simulink model "test_locked_rotor"  (R2025b)
settings: Solver=ode45  StartTime=0.0  StopTime=1  MaxStep=1e-4  RelTol=1e-6
undefined symbols (not defined in the file): D, D_p, F_load, L_lr, L_ls, Lm0, masa, Rr, Rs, tau_p, Tr_p, Vqs, we
settings Model: Creator=Lenovo  LastModifiedBy=LOQ

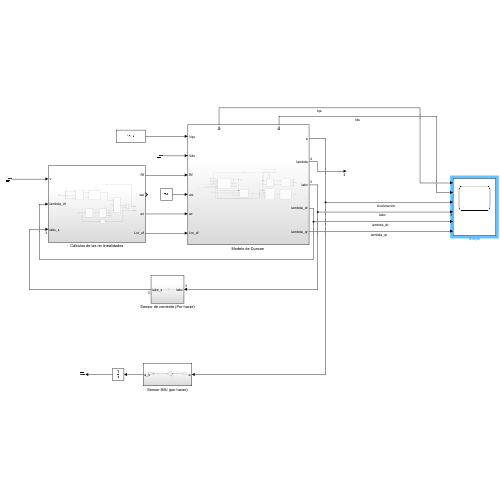
[thumbnail: Simulink's stored preview of the top-level diagram]
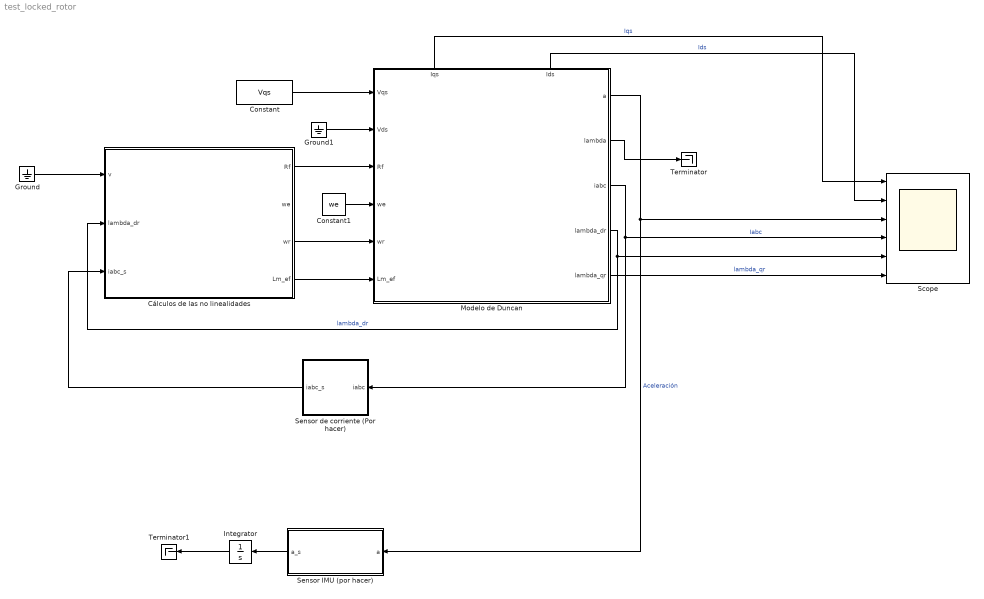
== system test_locked_rotor ==
  Constant : Constant  Value=Vqs
  Constant1 : Constant  Value=we
  Cálculos de las no linealidades : Subsystem
  Ground : Ground
  Ground1 : Ground
  Integrator : Integrator
  "Modelo de Duncan " : Subsystem
      settings: PortSchema="{\"entries\":[{\"content\":{\"sides\":[{\"content\":{\"connectorIds\":[\"In1\",\"In2\",\"In3\",\"In4\",\"In5\",\"In6\"]},\"type\":\"ConnectorPlacement.EquallySpacedRectSide\",\"uuid\":\"e25e1f22-370f-40c7-9e30-0a4cdda9d465\"},{\"content\":{\"connectorIds\":[\"Out1\",\"Out2\",\"Out3\",\"Out4\",\"Out5\"],\"side\":\"RIGHT\"},\"type\":\"ConnectorPlacement.EquallySpacedRectSide\",\"uuid\":\"8b806a62-390d-43d9-93c3-c856eeb20bab\"},{\"content\":{\"connectorIds\":[\"Out6\",\"Out7\"],\"side\":\"TOP\"},\"type\":\"ConnectorPlacement.EquallySpacedRectSide\",\"uuid\":\"b8ec9e8c-7518-4548-a43a-6e04a17b40db\"}]},\"type\":\"ConnectorPlacement.EquallySpacedConnector\",\"uuid\":\"66099662-dcc9-448a-97d1-76d3eb83184e\"}],\"packageUris\":[\"http://schema.mathworks.com/mf0/Connector/R2020b\"],\"version\":\"1.0\"}"
  Scope : Scope  NumInputPorts=6
      settings: ActiveDisplayYMinimum=-214.7307221633354  ActiveDisplayYMaximum=199.20639027449207
  Sensor IMU (por hacer) : Subsystem
  Sensor de corriente (Por hacer) : Subsystem
  Terminator : Terminator
  Terminator1 : Terminator
  wires:
  "Modelo de Duncan "/1(a) -> Sensor IMU (por hacer)/1(a), Scope/3  "Aceleración"
  Sensor IMU (por hacer)/1(a_s) -> Integrator/1
  "Modelo de Duncan "/3(iabc) -> Sensor de corriente (Por hacer)/1(iabc), Scope/4  "Iabc"
  Cálculos de las no linealidades/1(Rf) -> "Modelo de Duncan "/3(Rf)
  Cálculos de las no linealidades/3(wr) -> "Modelo de Duncan "/5(wr)
  Cálculos de las no linealidades/4(Lm_ef) -> "Modelo de Duncan "/6(Lm_ef)
  Sensor de corriente (Por hacer)/1(iabc_s) -> Cálculos de las no linealidades/3(iabc_s)
  "Modelo de Duncan "/2(lambda) -> Terminator/1
  "Modelo de Duncan "/4(lambda_dr) -> Cálculos de las no linealidades/2(lambda_dr), Scope/5  "lambda_dr"
  Integrator/1 -> Terminator1/1
  Ground/1 -> Cálculos de las no linealidades/1(v)
  Ground1/1 -> "Modelo de Duncan "/2(Vds)
  Constant/1 -> "Modelo de Duncan "/1(Vqs)
  Constant1/1 -> "Modelo de Duncan "/4(we)
  "Modelo de Duncan "/6(Iqs) -> Scope/1  "Iqs"
  "Modelo de Duncan "/7(Ids) -> Scope/2  "Ids"
  "Modelo de Duncan "/5(lambda_qr) -> Scope/6  "lambda_qr"

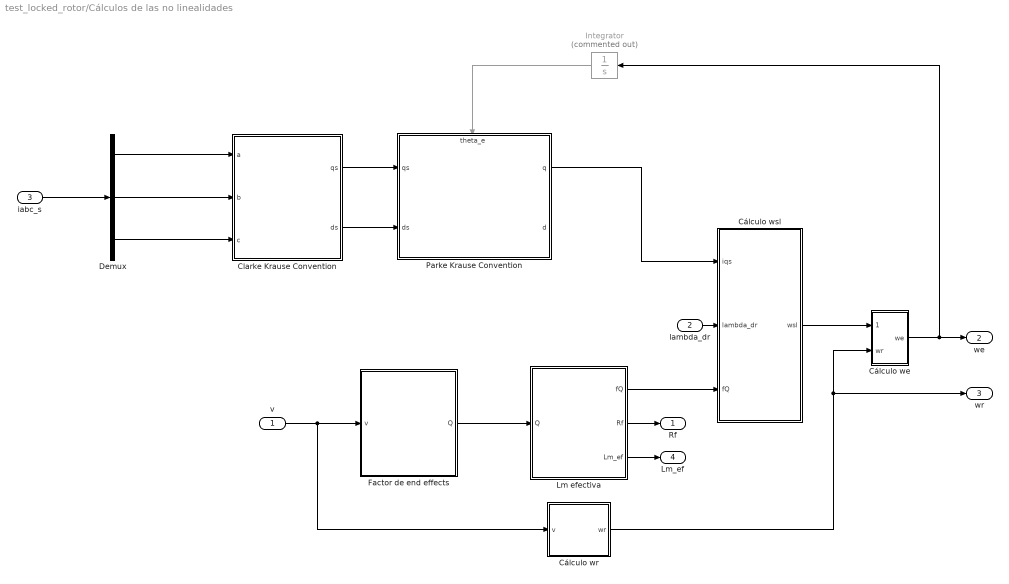
== system test_locked_rotor/Cálculos de las no linealidades ==
  v : Inport
  lambda_dr : Inport  Port=2
  iabc_s : Inport  Port=3
  Clarke Krause Convention : Subsystem
  Cálculo we : Subsystem
  Cálculo wr : Subsystem
  Cálculo wsl : Subsystem
  Demux : Demux  Outputs=3
  Factor de end effects : Subsystem
  Integrator : Integrator  Commented=on
  Lm efectiva : Subsystem
  Parke Krause Convention : Subsystem
      settings: PortSchema="{\"entries\":[{\"content\":{\"sides\":[{\"content\":{\"connectorIds\":[\"In1\",\"In2\"]},\"type\":\"ConnectorPlacement.EquallySpacedRectSide\",\"uuid\":\"727c49c2-322c-4428-ae94-4dccace1ba58\"},{\"content\":{\"connectorIds\":[\"Out1\",\"Out2\"],\"side\":\"RIGHT\"},\"type\":\"ConnectorPlacement.EquallySpacedRectSide\",\"uuid\":\"a4a3860a-23f1-45ee-a3a2-be69e979ab21\"},{\"content\":{\"connectorIds\":[\"In3\"],\"side\":\"TOP\"},\"type\":\"ConnectorPlacement.EquallySpacedRectSide\",\"uuid\":\"c36ae6a8-af84-4362-94ca-46fd0807c2cb\"}]},\"type\":\"ConnectorPlacement.EquallySpacedConnector\",\"uuid\":\"3c85f25c-260c-4438-9c99-6a3b31db29b6\"}],\"packageUris\":[\"http://schema.mathworks.com/mf0/Connector/R2020b\"],\"version\":\"1.0\"}"
  Rf : Outport
  we : Outport  Port=2
  wr : Outport  Port=3
  Lm_ef : Outport  Port=4
  wires:
  lambda_dr/1 -> Cálculo wsl/2(lambda_dr)
  Cálculo wr/1(wr) -> wr/1, Cálculo we/2(wr)
  Lm efectiva/1(fQ) -> Cálculo wsl/3(fQ)
  Factor de end effects/1(Q) -> Lm efectiva/1(Q)
  v/1 -> Cálculo wr/1(v), Factor de end effects/1(v)
  Cálculo we/1(we) -> Integrator/1, we/1
  Cálculo wsl/1(wsl) -> Cálculo we/1(wsl)
  Lm efectiva/3(Lm_ef) -> Lm_ef/1
  Lm efectiva/2(Rf) -> Rf/1
  Clarke Krause Convention/1(qs) -> Parke Krause Convention/1(qs)
  Clarke Krause Convention/2(ds) -> Parke Krause Convention/2(ds)
  Integrator/1 -> Parke Krause Convention/3(theta_e)
  Demux/1 -> Clarke Krause Convention/1(a)
  Demux/2 -> Clarke Krause Convention/2(b)
  Demux/3 -> Clarke Krause Convention/3(c)
  iabc_s/1 -> Demux/1
  Parke Krause Convention/1(q) -> Cálculo wsl/1(iqs)

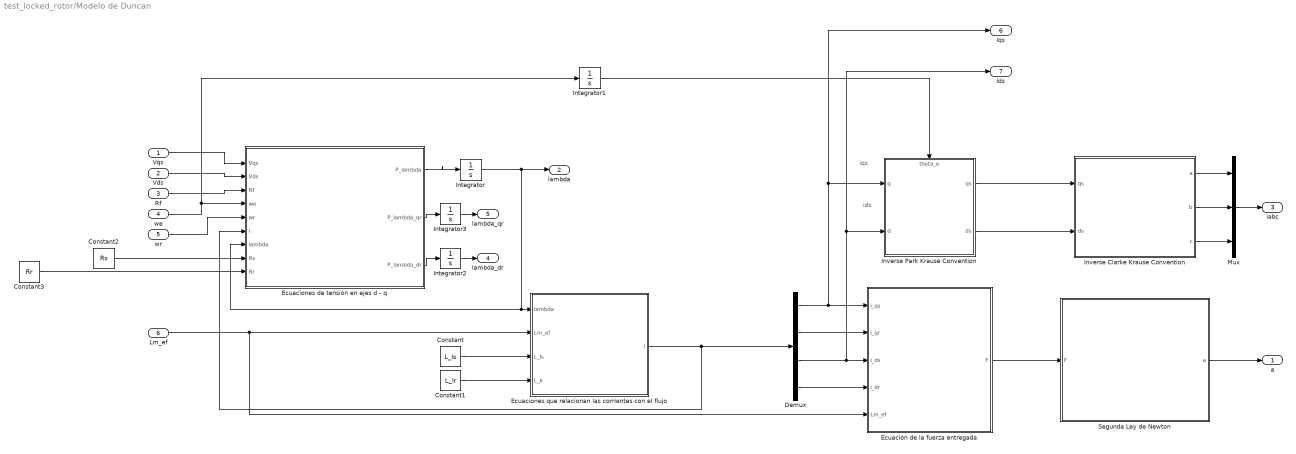
== system test_locked_rotor/Modelo de Duncan  ==
  note: ids
  note: iqs
  Vqs : Inport
  Vds : Inport  Port=2
  Rf : Inport  Port=3
  we : Inport  Port=4
  wr : Inport  Port=5
  Lm_ef : Inport  Port=6
  Constant : Constant  Value=L_ls
  Constant1 : Constant  Value=L_lr
  Constant2 : Constant  Value=Rs
  Constant3 : Constant  Value=Rr
  Demux : Demux
  Ecuaciones de tensión en ejes d - q : MATLAB Function  TreatAsAtomicUnit=on
  Ecuaciones que relacionan las corrientes con el flujo : MATLAB Function  TreatAsAtomicUnit=on
  Ecuación de la fuerza entregada : Subsystem
  Integrator : Integrator  InitialCondition=zeros(4,1)
  Integrator1 : Integrator
  Integrator2 : Integrator
  Integrator3 : Integrator
  Inverse Clarke Krause Convention : Subsystem
  Inverse Park Krause Convention : Subsystem
      settings: PortSchema="{\"entries\":[{\"content\":{\"sides\":[{\"content\":{\"connectorIds\":[\"In1\",\"In2\"]},\"type\":\"ConnectorPlacement.EquallySpacedRectSide\",\"uuid\":\"727c49c2-322c-4428-ae94-4dccace1ba58\"},{\"content\":{\"connectorIds\":[\"Out1\",\"Out2\"],\"side\":\"RIGHT\"},\"type\":\"ConnectorPlacement.EquallySpacedRectSide\",\"uuid\":\"a4a3860a-23f1-45ee-a3a2-be69e979ab21\"},{\"content\":{\"connectorIds\":[\"In3\"],\"side\":\"TOP\"},\"type\":\"ConnectorPlacement.EquallySpacedRectSide\",\"uuid\":\"c36ae6a8-af84-4362-94ca-46fd0807c2cb\"}]},\"type\":\"ConnectorPlacement.EquallySpacedConnector\",\"uuid\":\"3c85f25c-260c-4438-9c99-6a3b31db29b6\"}],\"packageUris\":[\"http://schema.mathworks.com/mf0/Connector/R2020b\"],\"version\":\"1.0\"}"
  Mux : Mux  Inputs=3
  Segunda Ley de Newton : Subsystem
  a : Outport
  lambda : Outport  Port=2
  iabc : Outport  Port=3
  lambda_dr : Outport  Port=4
  lambda_qr : Outport  Port=5
  Iqs : Outport  Port=6
  Ids : Outport  Port=7
  wires:
  we/1 -> Integrator1/1, Ecuaciones de tensión en ejes d - q/4(we)
  Ecuación de la fuerza entregada/1(F) -> Segunda Ley de Newton/1(F)
  Ecuaciones de tensión en ejes d - q/1(P_lambda) -> Integrator/1
  Vds/1 -> Ecuaciones de tensión en ejes d - q/2(Vds)
  Ecuaciones que relacionan las corrientes con el flujo/1(i) -> Ecuaciones de tensión en ejes d - q/6(i), Demux/1
  Integrator/1 -> Ecuaciones que relacionan las corrientes con el flujo/1(lambda), Ecuaciones de tensión en ejes d - q/7(lambda), lambda/1
  Constant1/1 -> Ecuaciones que relacionan las corrientes con el flujo/4(L_lr)
  Vqs/1 -> Ecuaciones de tensión en ejes d - q/1(Vqs)
  Constant/1 -> Ecuaciones que relacionan las corrientes con el flujo/3(L_ls)
  wr/1 -> Ecuaciones de tensión en ejes d - q/5(wr)
  Segunda Ley de Newton/1(a) -> a/1
  Rf/1 -> Ecuaciones de tensión en ejes d - q/3(Rf)
  Lm_ef/1 -> Ecuación de la fuerza entregada/5(Lm_ef), Ecuaciones que relacionan las corrientes con el flujo/2(Lm_ef)
  Inverse Park Krause Convention/2(ds) -> Inverse Clarke Krause Convention/2(ds)
  Inverse Park Krause Convention/1(qs) -> Inverse Clarke Krause Convention/1(qs)
  Integrator1/1 -> Inverse Park Krause Convention/3(theta_e)
  Inverse Clarke Krause Convention/1(a) -> Mux/1
  Inverse Clarke Krause Convention/2(b) -> Mux/2
  Inverse Clarke Krause Convention/3(c) -> Mux/3
  Mux/1 -> iabc/1
  Ecuaciones de tensión en ejes d - q/3(P_lambda_dr) -> Integrator2/1
  Integrator2/1 -> lambda_dr/1
  Integrator3/1 -> lambda_qr/1
  Ecuaciones de tensión en ejes d - q/2(P_lambda_qr) -> Integrator3/1
  Constant2/1 -> Ecuaciones de tensión en ejes d - q/8(Rs)
  Constant3/1 -> Ecuaciones de tensión en ejes d - q/9(Rr)
  Demux/1 -> Iqs/1, Inverse Park Krause Convention/1(q), Ecuación de la fuerza entregada/1(i_qs)
  Demux/2 -> Ecuación de la fuerza entregada/2(i_qr)
  Demux/3 -> Ids/1, Inverse Park Krause Convention/2(d), Ecuación de la fuerza entregada/3(i_ds)
  Demux/4 -> Ecuación de la fuerza entregada/4(i_dr)

== system test_locked_rotor/Sensor IMU (por hacer) ==
  a : Inport
  Gain : Gain
  a_s : Outport
  wires:
  Gain/1 -> a_s/1
  a/1 -> Gain/1

== system test_locked_rotor/Sensor de corriente (Por hacer) ==
  iabc : Inport
  Gain : Gain
  iabc_s : Outport
  wires:
  Gain/1 -> iabc_s/1
  iabc/1 -> Gain/1

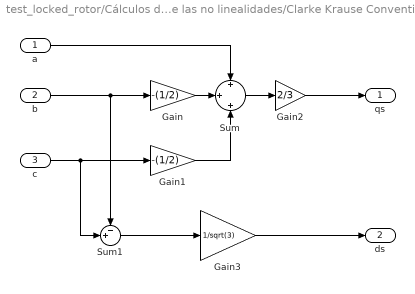
== system test_locked_rotor/Cálculos de las no linealidades/Clarke Krause Convention ==
  a : Inport
  b : Inport  Port=2
  c : Inport  Port=3
  Gain : Gain  Gain=-(1/2)
  Gain1 : Gain  Gain=-(1/2)
  Gain2 : Gain  Gain=2/3
  Gain3 : Gain  Gain=1/sqrt(3)
  Sum : Sum  Inputs=+|+|+
  Sum1 : Sum  Inputs=-+|
  qs : Outport
  ds : Outport  Port=2
  wires:
  b/1 -> Gain/1, Sum1/1
  Sum1/1 -> Gain3/1
  Sum/1 -> Gain2/1
  a/1 -> Sum/1
  Gain/1 -> Sum/2
  Gain3/1 -> ds/1
  Gain2/1 -> qs/1
  c/1 -> Sum1/2, Gain1/1
  Gain1/1 -> Sum/3

== system test_locked_rotor/Cálculos de las no linealidades/Cálculo we ==
  wsl : Inport
  wr : Inport  Port=2
  Sum : Sum  Inputs=|++
  we : Outport
  wires:
  Sum/1 -> we/1
  wsl/1 -> Sum/2
  wr/1 -> Sum/1

== system test_locked_rotor/Cálculos de las no linealidades/Cálculo wr ==
  v : Inport
  Gain : Gain  Gain=pi/tau_p
  wr : Outport
  wires:
  v/1 -> Gain/1
  Gain/1 -> wr/1

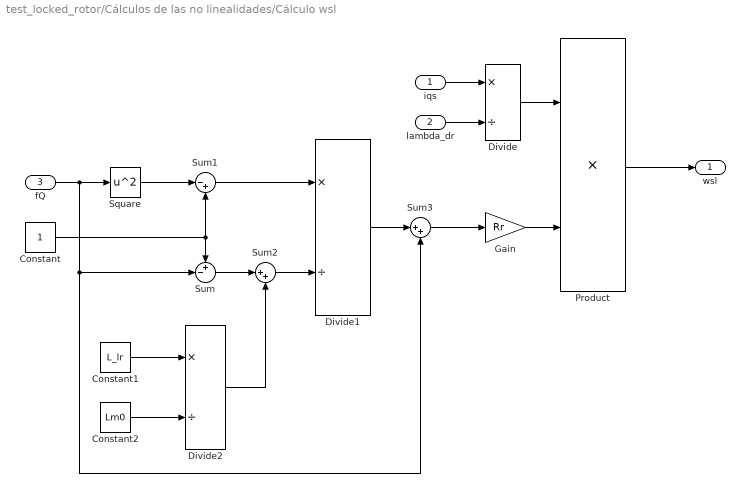
== system test_locked_rotor/Cálculos de las no linealidades/Cálculo wsl ==
  iqs : Inport
  lambda_dr : Inport  Port=2
  fQ : Inport  Port=3
  Constant : Constant
  Constant1 : Constant  Value=L_lr
  Constant2 : Constant  Value=Lm0
  Divide : Product  Inputs=*/
  Divide1 : Product  Inputs=*/
  Divide2 : Product  Inputs=*/
  Gain : Gain  Gain=Rr
  Product : Product
  Square : Math  Operator=square
  Sum : Sum  Inputs=+-|
  Sum1 : Sum  Inputs=|-+
  Sum2 : Sum  Inputs=|++
  Sum3 : Sum  Inputs=|++
  wsl : Outport
  wires:
  iqs/1 -> Divide/1
  lambda_dr/1 -> Divide/2
  Constant/1 -> Sum/1, Sum1/2
  fQ/1 -> Sum3/2, Sum/2, Square/1
  Square/1 -> Sum1/1
  Sum1/1 -> Divide1/1
  Constant1/1 -> Divide2/1
  Constant2/1 -> Divide2/2
  Sum/1 -> Sum2/1
  Sum2/1 -> Divide1/2
  Divide2/1 -> Sum2/2
  Divide1/1 -> Sum3/1
  Sum3/1 -> Gain/1
  Gain/1 -> Product/2
  Divide/1 -> Product/1
  Product/1 -> wsl/1

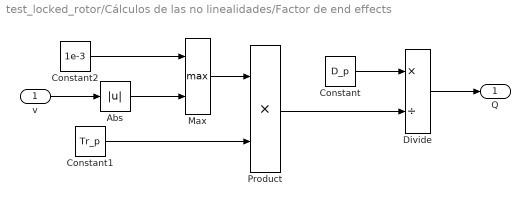
== system test_locked_rotor/Cálculos de las no linealidades/Factor de end effects ==
  v : Inport
  Abs : Abs  SaturateOnIntegerOverflow=off
  Constant : Constant  Value=D_p
  Constant1 : Constant  Value=Tr_p
  Constant2 : Constant  Value=1e-3
  Divide : Product  Inputs=*/
  Max : MinMax  Function=max  Inputs=2
  Product : Product
  Q : Outport
  wires:
  Constant/1 -> Divide/1
  Constant1/1 -> Product/2
  v/1 -> Abs/1
  Max/1 -> Product/1
  Abs/1 -> Max/2
  Constant2/1 -> Max/1
  Product/1 -> Divide/2
  Divide/1 -> Q/1

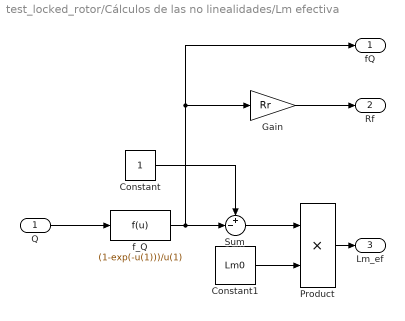
== system test_locked_rotor/Cálculos de las no linealidades/Lm efectiva ==
  Q : Inport
  Constant : Constant
  Constant1 : Constant  Value=Lm0
  Gain : Gain  Gain=Rr
  Product : Product
  Sum : Sum  Inputs=+-|
  f_Q : Fcn  Expr=(1-exp(-u(1)))/u(1)
  fQ : Outport
  Rf : Outport  Port=2
  Lm_ef : Outport  Port=3
  wires:
  Product/1 -> Lm_ef/1
  Sum/1 -> Product/1
  Constant1/1 -> Product/2
  f_Q/1 -> fQ/1, Gain/1, Sum/2
  Constant/1 -> Sum/1
  Q/1 -> f_Q/1
  Gain/1 -> Rf/1

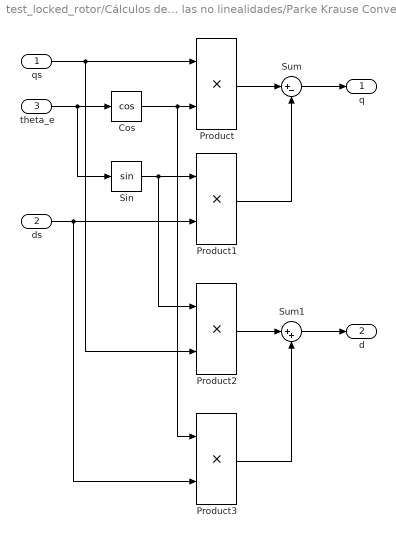
== system test_locked_rotor/Cálculos de las no linealidades/Parke Krause Convention ==
  qs : Inport
  ds : Inport  Port=2
  theta_e : Inport  Port=3
  Cos : Trigonometry  Operator=cos
  Product{,1..3} (4 alike) : Product
  Sin : Trigonometry
  Sum : Sum  Inputs=|+-
  Sum1 : Sum  Inputs=|++
  q : Outport
  d : Outport  Port=2
  wires:
  theta_e/1 -> Cos/1, Sin/1
  Product/1 -> Sum/1
  Product3/1 -> Sum1/2
  ds/1 -> Product3/2, Product1/2
  Cos/1 -> Product3/1, Product/2
  Product1/1 -> Sum/2
  qs/1 -> Product2/2, Product/1
  Sin/1 -> Product2/1, Product1/1
  Sum1/1 -> d/1
  Product2/1 -> Sum1/1
  Sum/1 -> q/1

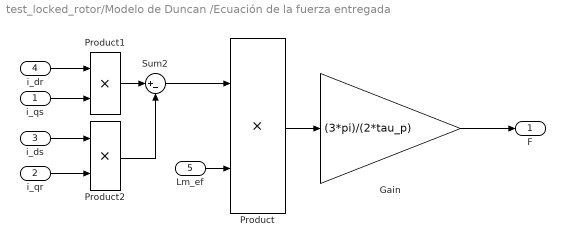
== system test_locked_rotor/Modelo de Duncan /Ecuación de la fuerza entregada ==
  i_qs : Inport
  i_qr : Inport  Port=2
  i_ds : Inport  Port=3
  i_dr : Inport  Port=4
  Lm_ef : Inport  Port=5
  Gain : Gain  Gain=(3*pi)/(2*tau_p)
  Product : Product
  Product1 : Product
  Product2 : Product
  Sum2 : Sum  Inputs=|+-
  F : Outport
  wires:
  Product/1 -> Gain/1
  Lm_ef/1 -> Product/2
  Gain/1 -> F/1
  Product1/1 -> Sum2/1
  Product2/1 -> Sum2/2
  i_ds/1 -> Product2/1
  Sum2/1 -> Product/1
  i_qr/1 -> Product2/2
  i_qs/1 -> Product1/2
  i_dr/1 -> Product1/1

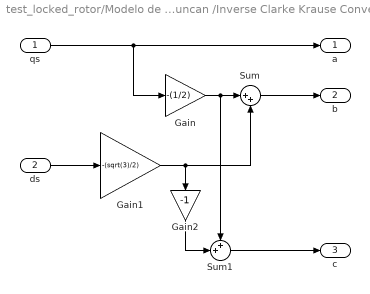
== system test_locked_rotor/Modelo de Duncan /Inverse Clarke Krause Convention ==
  qs : Inport
  ds : Inport  Port=2
  Gain : Gain  Gain=-(1/2)
  Gain1 : Gain  Gain=-(sqrt(3)/2)
  Gain2 : Gain  Gain=-1
  Sum : Sum  Inputs=|++
  Sum1 : Sum  Inputs=++|
  a : Outport
  b : Outport  Port=2
  c : Outport  Port=3
  wires:
  qs/1 -> a/1, Gain/1
  Gain2/1 -> Sum1/2
  Gain/1 -> Sum/1, Sum1/1
  Gain1/1 -> Gain2/1, Sum/2
  Sum/1 -> b/1
  ds/1 -> Gain1/1
  Sum1/1 -> c/1

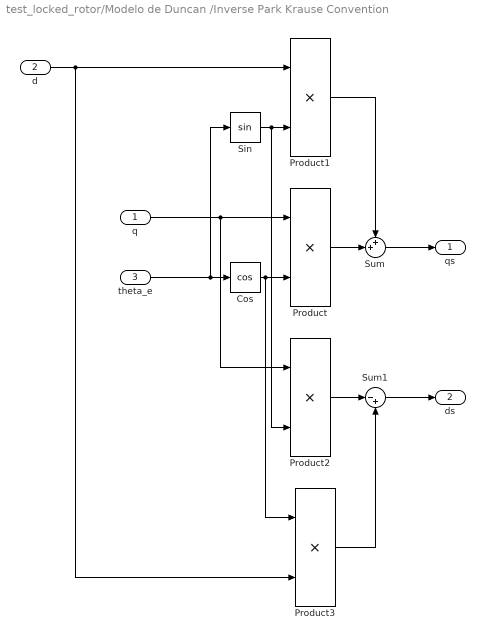
== system test_locked_rotor/Modelo de Duncan /Inverse Park Krause Convention ==
  q : Inport
  d : Inport  Port=2
  theta_e : Inport  Port=3
  Cos : Trigonometry  Operator=cos
  Product{,1..3} (4 alike) : Product
  Sin : Trigonometry
  Sum : Sum  Inputs=++|
  Sum1 : Sum  Inputs=|-+
  qs : Outport
  ds : Outport  Port=2
  wires:
  Cos/1 -> Product3/1, Product/2
  theta_e/1 -> Sin/1, Cos/1
  q/1 -> Product2/1, Product/1
  Product1/1 -> Sum/1
  Sum/1 -> qs/1
  Product/1 -> Sum/2
  Sin/1 -> Product2/2, Product1/2
  d/1 -> Product3/2, Product1/1
  Product2/1 -> Sum1/1
  Product3/1 -> Sum1/2
  Sum1/1 -> ds/1

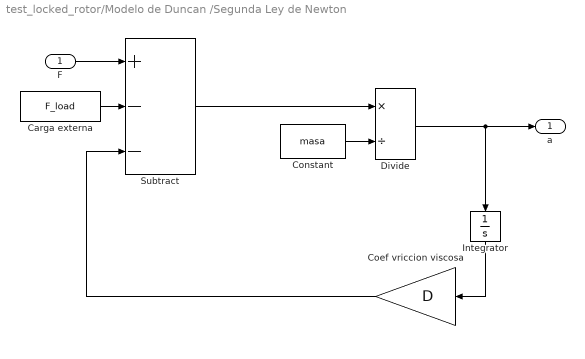
== system test_locked_rotor/Modelo de Duncan /Segunda Ley de Newton ==
  F : Inport
  Carga externa : Constant  Value=F_load
  Coef vriccion viscosa : Gain  Gain=D
  Constant : Constant  Value=masa
  Divide : Product  Inputs=*/
  Integrator : Integrator
  Subtract : Sum  Inputs=+--
  a : Outport
  wires:
  Integrator/1 -> Coef vriccion viscosa/1
  F/1 -> Subtract/1
  Coef vriccion viscosa/1 -> Subtract/3
  Carga externa/1 -> Subtract/2
  Subtract/1 -> Divide/1
  Divide/1 -> a/1, Integrator/1
  Constant/1 -> Divide/2

== matlab function test_locked_rotor/Modelo de Duncan /Ecuaciones que relacionan las corrientes con el flujo ==
  data: i output; lambda input; Lm_ef input; L_ls input; L_lr input

function i = fcn(lambda,Lm_ef,L_ls,L_lr)

    % Definición de los vectores de estado

    %i = [iqs,iqr,ids,idr]';
    %lambda = [lambda_qs,lambda_qr,lambda_ds,lambda_dr]'; 

    L1 = [(L_ls+Lm_ef),Lm_ef;Lm_ef,(L_lr+Lm_ef)];
    L1_inv = inv(L1);

    L2_inv = L1_inv;

    L_inv = [L1_inv,zeros(2);zeros(2),L2_inv];

    % Ecuación final que relaciona lambda con i

    i = L_inv*lambda;

== matlab function test_locked_rotor/Modelo de Duncan /Ecuaciones de tensión en ejes d - q ==
  data: Vqs input; P_lambda output; P_lambda_qr output; Vds input; Rf input; we input; wr input; i input; lambda input; P_lambda_dr output; Rs input; Rr input
function [P_lambda,P_lambda_qr,P_lambda_dr]  = fcn(Vqs,Vds,Rf,we,wr,i,lambda,Rs,Rr)

% Ecuación cuasi-lineal a representar (con estados)

% der lambda = V + R*i + w*lambda

% Definición de los vectores de estado 

V = [Vqs 0 Vds 0]';

% iqs = i(1,1);
% iqr = i(1,2);
% ids = i(1,3);
% idr = i(1,4);
% i = [iqs,iqr,ids,idr]';
% 
% lambda_qs = lambda(1);
% lambda_qr = lambda(2);
% lambda_ds = lambda(3);
% lambda_dr = lambda(4);
% 
% lambda = [lambda_qs,lambda_qr,lambda_ds,lambda_dr]';

% Definición de las matrices 

R1 = [-(Rs+Rf) -Rf; -Rf -(Rr+Rf)];
R2 = R1;
R = [R1 zeros(2);zeros(2) R2];

w1 = [-we 0;0 -(we-wr)];
w2 = [we 0;0 (we-wr)];
w = [zeros(2) w1; w2 zeros(2)];

% Ecuación final

P_lambda = V + R*i + w*lambda;

% Flujos q y d del principal (s = el que alimentamos) y secundario (r =
% placa)


P_lambda_qr = P_lambda(2);
P_lambda_dr = P_lambda(4);
